simulink model "model"  (R2026b)
settings: Solver=VariableStepAuto  StopTime=5.5  FixedStep=0.0001
InitFcn:
  | init_vehicle;
values from neighbouring files (symbols this model uses):
  vehicle = Simulink.Parameter(vehicle)    [fit_log.m]    (also in init_vehicle.m)
undefined symbols (not defined in the file or in its folder): b6bc
libraries: simulink x2, slpidlib x1
settings Model: Creator=Madelyn  LastModifiedBy=Madelyn
settings RTWCC: GPUComputeCapability=5.0

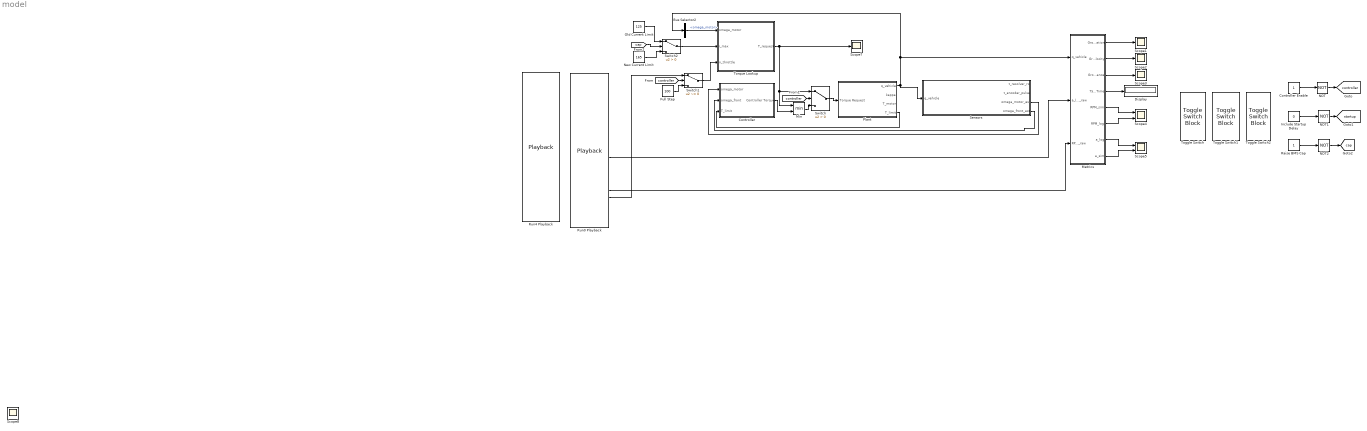
== system model ==
  Bus Selector2 : BusSelector  OutputSignals=omega_motor
  Controller : Subsystem
  Controller Enable : Constant
  Display : Display
  Full Step : Constant  Value=100
  Include Startup Delay : Constant  Value=0
  Metrics : Subsystem
  Min : MinMax  Inputs=2
  NOT : Logic  Operator=NOT  IconShape=distinctive  AllPortsSameDT=off  OutDataTypeStr=boolean
  NOT1 : Logic  Operator=NOT  IconShape=distinctive  AllPortsSameDT=off  OutDataTypeStr=boolean
  NOT2 : Logic  Operator=NOT  IconShape=distinctive  AllPortsSameDT=off  OutDataTypeStr=boolean
  New Current Limit : Constant  Value=165
  Old Current Limit : Constant  Value=125
  Plant : Subsystem
  Raise BMS Cap : Constant
  Run0 Playback : Playback  NumPorts=35  PartName=7320df4f-afde-441e-80d8-dbf4e5708069  TablePosition=Bottom
  Run4 Playback : Playback  NumPorts=35  PartName=9ae1c79e-69de-485c-b6bc-1278a8bcc222  TablePosition=Bottom
  Scope{1..3,7..8} (5 alike) : Scope
      Scope1 settings: ActiveDisplayYMinimum=-1.0070209667799948  ActiveDisplayYMaximum=9.0631887010199552
      Scope2 settings: ActiveDisplayYMinimum=-4.8200936981689466  ActiveDisplayYMaximum=37.977704065737591  DataLoggingVariableName=ScopeData3
      Scope3 settings: DataLoggingVariableName=ScopeData5
      Scope7 settings: ActiveDisplayYMinimum=100.18093555938822  ActiveDisplayYMaximum=233.31322938229022  DataLoggingVariableName=ScopeData11
      Scope8 settings: ActiveDisplayYMinimum=-12.499999999999996  ActiveDisplayYMaximum=112.5  DataLoggingVariableName=ScopeData9
  Scope4 : Scope  NumInputPorts=2
      settings: DataLoggingVariableName=ScopeData7
  Scope5 : Scope  NumInputPorts=2
      settings: DataLoggingVariableName=ScopeData8
  Sensors : Subsystem
  Switch : Switch  Criteria=u2 > Threshold  SaturateOnIntegerOverflow=off  InputSameDT=off
  Switch1 : Switch  Criteria=u2 ~= 0  SaturateOnIntegerOverflow=off  InputSameDT=off
  Switch2 : Switch  Criteria=u2 > Threshold  SaturateOnIntegerOverflow=off  InputSameDT=off
  Toggle Switch : ToggleSwitchBlock
  Toggle Switch1 : ToggleSwitchBlock
  Toggle Switch2 : ToggleSwitchBlock
  Torque Lookup : MATLAB Function  TreatAsAtomicUnit=on
  tag scope: cap=global, controller=global, startup=global
  wires:
  Sensors/3(omega_motor_est) -> Controller/1(omega_motor)
  Sensors/4(omega_front_est) -> Controller/2(omega_front)
  Plant/1(q_vehicle) -> Sensors/1(q_vehicle), Bus Selector2/1, Metrics/1(q_vehicle)
  Bus Selector2/1 -> Torque Lookup/1(omega_motor)  "<omega_motor>"
  Run0 Playback/20 -> Metrics/2(a_log_raw)
  Run0 Playback/29 -> Metrics/3(RPM_log_raw)
  Torque Lookup/1(T_request) -> Scope7/1, Min/1, Switch/1
  Run0 Playback/31 -> Switch1/1
  Min/1 -> Switch/3
  Full Step/1 -> Switch1/3
  Switch1/1 -> Torque Lookup/3(n_throttle)
  Controller Enable/1 -> NOT/1
  [controller] -> Switch1/2
  [controller] -> Switch/2
  NOT/1 -> [controller]
  Include Startup Delay/1 -> NOT1/1
  NOT1/1 -> [startup]
  Raise BMS Cap/1 -> NOT2/1
  NOT2/1 -> [cap]
  Old Current Limit/1 -> Switch2/1
  Switch2/1 -> Torque Lookup/2(i_max)
  New Current Limit/1 -> Switch2/3
  [cap] -> Switch2/2
  Metrics/1(Ground Acceleration) -> Scope1/1
  Metrics/2(Ground Velocity) -> Scope2/1
  Metrics/3(Ground Distance) -> Scope3/1
  Metrics/4(75m Time) -> Display/1
  Metrics/5(RPM_sim) -> Scope4/1
  Metrics/6(RPM_log) -> Scope4/2
  Metrics/7(a_log) -> Scope5/1
  Metrics/8(a_sim) -> Scope5/2
  Controller/1(Controller Torque) -> Min/2
  Plant/4(T_limit) -> Controller/3(T_limit)
  Switch/1 -> Plant/1(Torque Request)

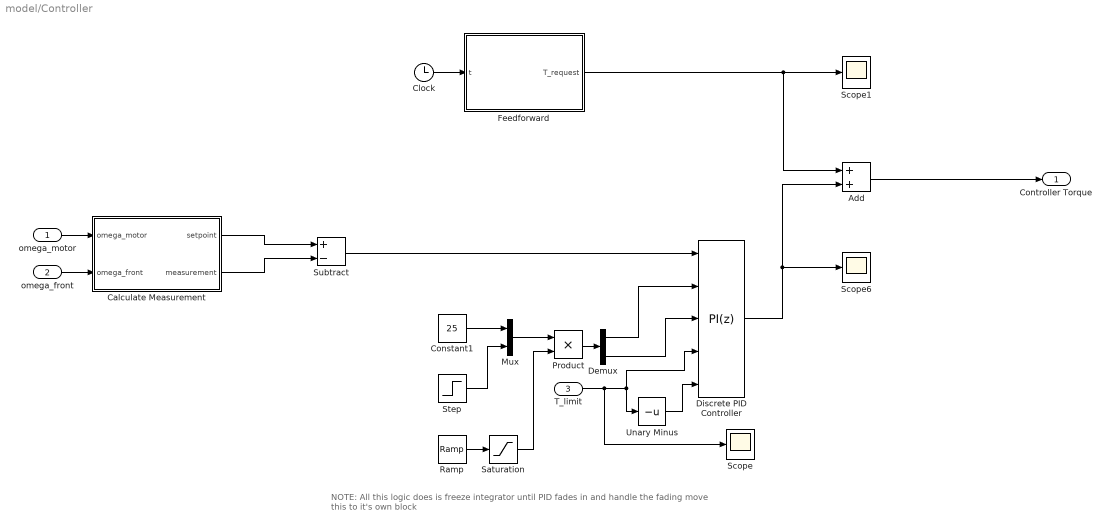
== system model/Controller ==
  note: NOTE: All this logic does is freeze integrator until PID fades in and handle the fading
      | move this to it's own block
  omega_motor : Inport
  omega_front : Inport  Port=2
  T_limit : Inport  Port=3
  Add : Sum
  Calculate Measurement : MATLAB Function  TreatAsAtomicUnit=on
  Clock : Clock
  Constant1 : Constant  Value=25
  Demux : Demux  Outputs=2
  Discrete PID Controller : slpidlib/PID Controller  Controller=PI  Form=Parallel  TimeDomain=Discrete-time  UseExternalTs=off  SampleTime=0.003  IntegratorMethod=Forward Euler  FilterMethod=Forward Euler  ControllerParametersSource=external  P=50  I=400  UseKiTs=off  D=0  UseExternalDerivativeSource=off  N=100  UseFilter=on  TunerSelectOption=Transfer Function Based (PID Tuner App)  InitialConditionSource=internal  InitialConditionForIntegrator=0  InitialConditionForFilter=0  DifferentiatorICPrevScaledInput=0  ExternalReset=none  TrackingMode=off  Kt=1  LimitOutput=on  SatLimitsSource=external  UpperSaturationLimit=inf  LowerSaturationLimit=-inf  LinearizeAsGain=off  AntiWindupMode=clamping  Kb=1  LimitIntegrator=on  UpperIntegratorSaturationLimit=180  LowerIntegratorSaturationLimit=-180  POutMin=[]  POutMax=[]  IOutMin=[]  IOutMax=[]  DOutMin=[]  DOutMax=[]  NOutMin=[]  NOutMax=[]  SumOutMin=[]  SumOutMax=[]  SaturationOutMin=[]  SaturationOutMax=[]  PParamMin=[]  PParamMax=[]  IParamMin=[]  IParamMax=[]  DParamMin=[]  DParamMax=[]  NParamMin=[]  NParamMax=[]  KbParamMin=[]  KbParamMax=[]  KtParamMin=[]  KtParamMax=[]  KbOutMin=[]  KbOutMax=[]  KtOutMin=[]  KtOutMax=[]  IntegratorOutMin=[]  IntegratorOutMax=[]  FilterOutMin=[]  FilterOutMax=[]  SumI1OutMin=[]  SumI1OutMax=[]  SumI2OutMin=[]  SumI2OutMax=[]  SumI3OutMin=[]  SumI3OutMax=[]  SumI4OutMin=[]  SumI4OutMax=[]  SumDOutMin=[]  SumDOutMax=[]  DifferentiatorOutMin=[]  DifferentiatorOutMax=[]  FilterDiffOutCoefMin=[]  FilterDiffOutCoefMax=[]  ReciprocalOutMin=[]  ReciprocalOutMax=[]  SumDenOutMin=[]  SumDenOutMax=[]  SumNumOutMin=[]  SumNumOutMax=[]  DivideOutMin=[]  DivideOutMax=[]  UdiffTsProdOutMin=[]  UdiffTsProdOutMax=[]  NTsProdOutMin=[]  NTsProdOutMax=[]  UintegralTsProdOutMin=[]  UintegralTsProdOutMax=[]  UngainTsProdOutMin=[]  UngainTsProdOutMax=[]  ClampingZeroOutDataTypeStr=Inherit: Inherit via back propagation  ClampingZeroOutMin=[]  ClampingZeroOutMax=[]  FilterDenConstantOutDataTypeStr=Inherit: Inherit via back propagation  FilterDenConstantOutMin=[]  FilterDenConstantOutMax=[]  PCopyOutDataTypeStr=Inherit: Inherit via back propagation  PCopyOutMin=[]  PCopyOutMax=[]  NCopyOutDataTypeStr=Inherit: Inherit via back propagation  NCopyOutMin=[]  NCopyOutMax=[]  IntegratorContinuousStateAttributes=''  IntegratorStateMustResolveToSignalObject=off  IntegratorRTWStateStorageClass=Auto  FilterContinuousStateAttributes=''  FilterStateMustResolveToSignalObject=off  FilterRTWStateStorageClass=Auto  ParallelPVariant=ExternalParameters  IdealPVariant=Disabled  IVariant=ExternalParameters  DVariant=Disabled  IntegratorVariant=Discrete  SatVariant=External  AWVariant=DiscClampingParallel  PCopyVariant=Disabled  TRVariant=Disabled  FdbkBlocksVariant=Forward  IdealPFdbkVariant=Disabled  SatFdbkVariant=Disabled  DerivativeFilterVariant=Disabled  NVariant=Disabled  NCopyVariant=Disabled_SignalSpec  FilterICVariant=Disabled  IntegratorICVariant=InternalICs  ExternalResetVariant=Disabled  TRSumVariant=Passthrough  SumFdbkVariant=Disabled  SumVariant=Sum_PI  TsampFilterVariant=InternalTs  TsampNgainVariant=Passthrough  TsampIntegralVariant=Disabled_SignalSpec  ExternalSaturationOutDataTypeStr=Inherit: Same as second input  DerivativeSourceVariant=Disabled  PreIntVariant=InternalPreInt
      settings: LibrarySourceBlock=simulink/Discrete/Discrete PID Controller
  Feedforward : MATLAB Function  TreatAsAtomicUnit=on
  Mux : Mux  Inputs=2
  Product : Product
  Ramp : simulink/Sources/Ramp  slope=4  start=0.5  InitialOutput=0
  Saturation : Saturate  UpperLimit=1  LowerLimit=0
  Scope : Scope
      settings: ActiveDisplayYMinimum=130.59305560506354  ActiveDisplayYMaximum=189.48966048832625  DataLoggingVariableName=ScopeData16
  Scope1 : Scope
      settings: ActiveDisplayYMinimum=-19.769298544681185  ActiveDisplayYMaximum=177.9236869021307
  Scope6 : Scope
      settings: ActiveDisplayYMinimum=-24.158543429115252  ActiveDisplayYMaximum=189.40218177528487  DataLoggingVariableName=ScopeData6
  Step : Step  Time=0.5  FinalValue=250  SampleTime=0
  Subtract : Sum  Inputs=+-
  Unary Minus : UnaryMinus
  Controller Torque : Outport
  wires:
  Ramp/1 -> Saturation/1
  Mux/1 -> Product/1
  Constant1/1 -> Mux/1
  Product/1 -> Demux/1
  Saturation/1 -> Product/2
  Feedforward/1(T_request) -> Add/1, Scope1/1
  Step/1 -> Mux/2
  Demux/1 -> Discrete PID Controller/2
  Demux/2 -> Discrete PID Controller/3
  Add/1 -> Controller Torque/1
  T_limit/1 -> Scope/1, Unary Minus/1, Discrete PID Controller/4
  Unary Minus/1 -> Discrete PID Controller/5
  Discrete PID Controller/1 -> Scope6/1, Add/2
  omega_motor/1 -> Calculate Measurement/1(omega_motor)
  omega_front/1 -> Calculate Measurement/2(omega_front)
  Subtract/1 -> Discrete PID Controller/1
  Calculate Measurement/1(setpoint) -> Subtract/1
  Calculate Measurement/2(measurement) -> Subtract/2
  Clock/1 -> Feedforward/1(t)

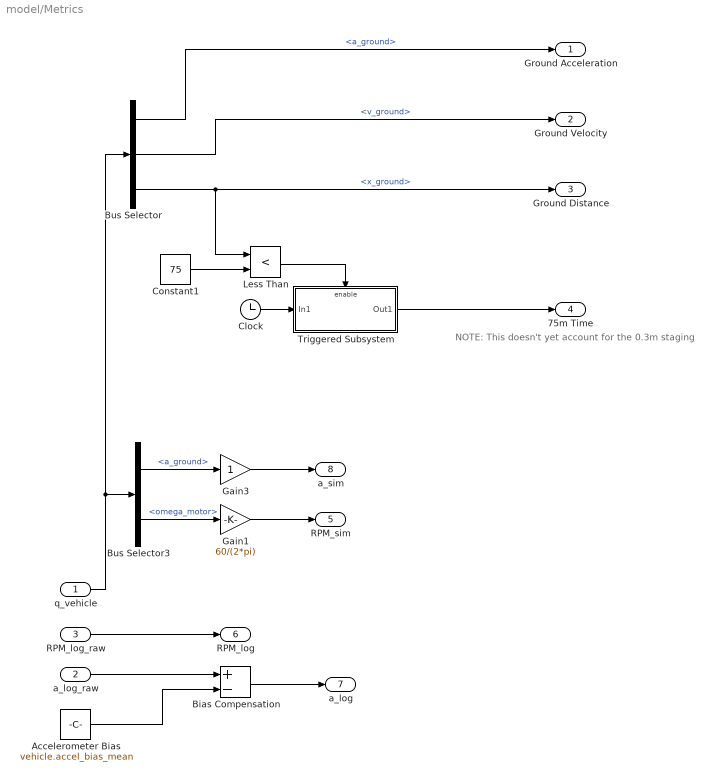
== system model/Metrics ==
  note: NOTE: This doesn't yet account for the 0.3m staging
  q_vehicle : Inport
  a_log_raw : Inport  Port=2
  RPM_log_raw : Inport  Port=3
  Accelerometer Bias : Constant  Value=vehicle.accel_bias_mean
  Bias Compensation : Sum  Inputs=+-
  Bus Selector : BusSelector  OutputSignals=a_ground,v_ground,x_ground
  Bus Selector3 : BusSelector  OutputSignals=a_ground,omega_motor
  Clock : Clock
  Constant1 : Constant  Value=75
  Gain1 : Gain  Gain=60/(2*pi)
  Gain3 : Gain
  Less Than : RelationalOperator  Operator=<  OutDataTypeStr=boolean  RndMeth=Simplest  InputSameDT=off
  Triggered Subsystem : Subsystem  TreatAsAtomicUnit=on
  Ground Acceleration : Outport
  Ground Velocity : Outport  Port=2
  Ground Distance : Outport  Port=3
  75m Time : Outport  Port=4
  RPM_sim : Outport  Port=5
  RPM_log : Outport  Port=6
  a_log : Outport  Port=7
  a_sim : Outport  Port=8
  wires:
  RPM_log_raw/1 -> RPM_log/1
  Accelerometer Bias/1 -> Bias Compensation/2
  a_log_raw/1 -> Bias Compensation/1
  Bus Selector3/1 -> Gain3/1  "<a_ground>"
  Gain1/1 -> RPM_sim/1
  q_vehicle/1 -> Bus Selector/1, Bus Selector3/1
  Bus Selector/2 -> Ground Velocity/1  "<v_ground>"
  Constant1/1 -> Less Than/2
  Less Than/1 -> Triggered Subsystem/Enable
  Bus Selector/3 -> Ground Distance/1, Less Than/1  "<x_ground>"
  Clock/1 -> Triggered Subsystem/1(In1)
  Bus Selector/1 -> Ground Acceleration/1  "<a_ground>"
  Bus Selector3/2 -> Gain1/1  "<omega_motor>"
  Triggered Subsystem/1(Out1) -> 75m Time/1
  Bias Compensation/1 -> a_log/1
  Gain3/1 -> a_sim/1

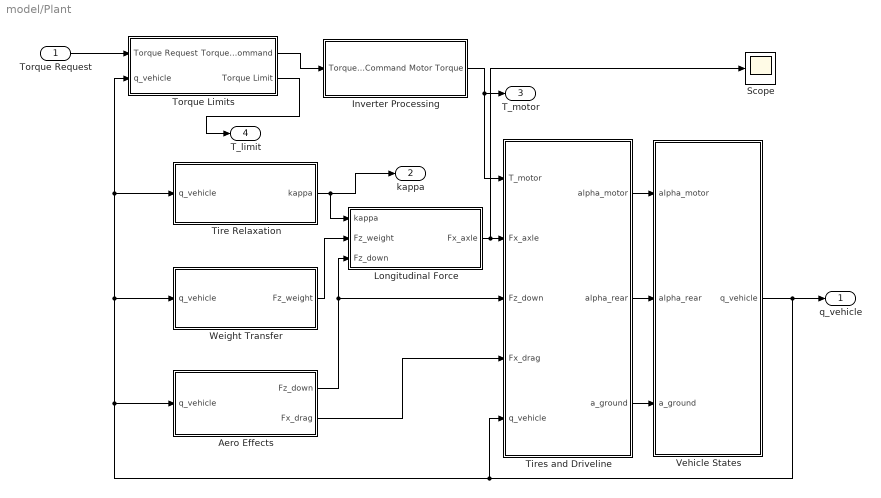
== system model/Plant ==
  Torque Request : Inport
  Aero Effects : Subsystem
  Inverter Processing : Subsystem
  Longitudinal Force : Subsystem
  Scope : Scope
      settings: ActiveDisplayYMinimum=-349.40408874349123  ActiveDisplayYMaximum=3144.6367986914215  DataLoggingVariableName=ScopeData4
  Tire Relaxation : Subsystem
  Tires and Driveline : Subsystem
  Torque Limits : Subsystem
  Vehicle States : Subsystem
  Weight Transfer : Subsystem
  q_vehicle : Outport
  kappa : Outport  Port=2
  T_motor : Outport  Port=3
  T_limit : Outport  Port=4
  wires:
  Tires and Driveline/3(a_ground) -> Vehicle States/3(a_ground)
  Vehicle States/1(q_vehicle) -> Tire Relaxation/1(q_vehicle), Torque Limits/2(q_vehicle), Weight Transfer/1(q_vehicle), Aero Effects/1(q_vehicle), Tires and Driveline/5(q_vehicle), q_vehicle/1
  Tires and Driveline/2(alpha_rear) -> Vehicle States/2(alpha_rear)
  Tires and Driveline/1(alpha_motor) -> Vehicle States/1(alpha_motor)
  Torque Limits/1(Torque Command) -> Inverter Processing/1(Torque Command)
  Tire Relaxation/1(kappa) -> kappa/1, Longitudinal Force/1(kappa)
  Weight Transfer/1(Fz_weight) -> Longitudinal Force/2(Fz_weight)
  Longitudinal Force/1(Fx_axle) -> Scope/1, Tires and Driveline/2(Fx_axle)
  Inverter Processing/1(Motor Torque) -> T_motor/1, Tires and Driveline/1(T_motor)
  Torque Request/1 -> Torque Limits/1(Torque Request)
  Torque Limits/2(Torque Limit) -> T_limit/1
  Aero Effects/2(Fx_drag) -> Tires and Driveline/4(Fx_drag)
  Aero Effects/1(Fz_down) -> Tires and Driveline/3(Fz_down), Longitudinal Force/3(Fz_down)

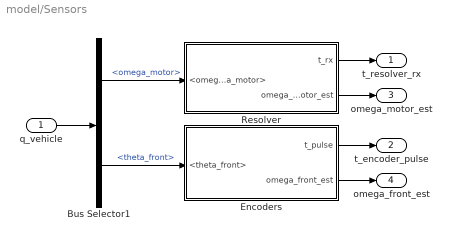
== system model/Sensors ==
  q_vehicle : Inport
  Bus Selector1 : BusSelector  OutputSignals=omega_motor,theta_front
  Encoders : Subsystem
  Resolver : Subsystem
  t_resolver_rx : Outport
  t_encoder_pulse : Outport  Port=2
  omega_motor_est : Outport  Port=3
  omega_front_est : Outport  Port=4
  wires:
  Bus Selector1/2 -> Encoders/1(<theta_front>)  "<theta_front>"
  q_vehicle/1 -> Bus Selector1/1
  Bus Selector1/1 -> Resolver/1(<omega_motor>)  "<omega_motor>"
  Resolver/1(t_rx) -> t_resolver_rx/1
  Resolver/2(omega_motor_est) -> omega_motor_est/1
  Encoders/1(t_pulse) -> t_encoder_pulse/1
  Encoders/2(omega_front_est) -> omega_front_est/1

== system model/Metrics/Triggered Subsystem ==
  In1 : Inport
  Enable : EnablePort
  Out1 : Outport
  wires:
  In1/1 -> Out1/1

== system model/Plant/Aero Effects ==
  q_vehicle : Inport
  Aero Effects : MATLAB Function  TreatAsAtomicUnit=on
  Bus Selector : BusSelector  OutputSignals=v_ground
  Fz_down : Outport
  Fx_drag : Outport  Port=2
  wires:
  Bus Selector/1 -> Aero Effects/1(v_ground)  "<v_ground>"
  q_vehicle/1 -> Bus Selector/1
  Aero Effects/1(Fz_down) -> Fz_down/1
  Aero Effects/2(Fx_drag) -> Fx_drag/1

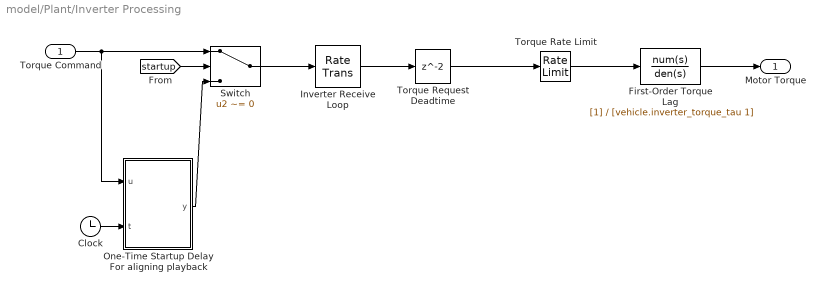
== system model/Plant/Inverter Processing ==
  Torque Command : Inport
  Clock : Clock
  First-Order Torque Lag : TransferFcn  Denominator=[vehicle.inverter_torque_tau 1]
  Inverter Receive Loop : RateTransition  OutPortSampleTime=vehicle.inverter_receive_period
  One-Time Startup Delay For aligning playback : MATLAB Function  TreatAsAtomicUnit=on
  Switch : Switch  Criteria=u2 ~= 0  SaturateOnIntegerOverflow=off  InputSameDT=off
  Torque Rate Limit : RateLimiter  RisingSlewLimit=vehicle.torque_rate_limit  FallingSlewLimit=-vehicle.torque_rate_limit  SampleTimeMode=inherited
  Torque Request Deadtime : Delay  SampleTime=vehicle.inverter_request_deadtime
  Motor Torque : Outport
  wires:
  Torque Rate Limit/1 -> First-Order Torque Lag/1
  Inverter Receive Loop/1 -> Torque Request Deadtime/1
  First-Order Torque Lag/1 -> Motor Torque/1
  Torque Request Deadtime/1 -> Torque Rate Limit/1
  Clock/1 -> One-Time Startup Delay For aligning playback/2(t)
  Torque Command/1 -> One-Time Startup Delay For aligning playback/1(u), Switch/1
  One-Time Startup Delay For aligning playback/1(y) -> Switch/3
  Switch/1 -> Inverter Receive Loop/1
  [startup] -> Switch/2

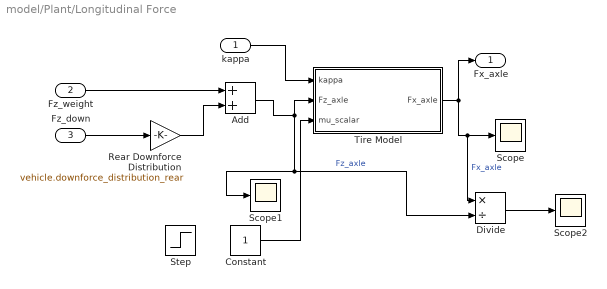
== system model/Plant/Longitudinal Force ==
  kappa : Inport
  Fz_weight : Inport  Port=2
  Fz_down : Inport  Port=3
  Add : Sum
  Constant : Constant
  Divide : Product  Inputs=*/
  "Rear Downforce Distribution " : Gain  Gain=vehicle.downforce_distribution_rear
  Scope : Scope
      settings: ActiveDisplayYMinimum=-328.964155800479  ActiveDisplayYMaximum=2960.6774022043114  DataLoggingVariableName=ScopeData13
  Scope1 : Scope
      settings: ActiveDisplayYMinimum=1302.8307308940846  ActiveDisplayYMaximum=2187.5559219532392  DataLoggingVariableName=ScopeData14
  Scope2 : Scope
      settings: ActiveDisplayYMinimum=-0.1766422510137696  ActiveDisplayYMaximum=1.5897802591239265  DataLoggingVariableName=ScopeData15
  Step : Step  Time=1.5  InitialValue=1  FinalValue=0.8  SampleTime=0
  Tire Model : MATLAB Function  TreatAsAtomicUnit=on
  Fx_axle : Outport
  wires:
  Fz_down/1 -> "Rear Downforce Distribution "/1
  kappa/1 -> Tire Model/1(kappa)
  Add/1 -> Divide/2, Scope1/1, Tire Model/2(Fz_axle)  "Fz_axle"
  Fz_weight/1 -> Add/1
  "Rear Downforce Distribution "/1 -> Add/2
  Tire Model/1(Fx_axle) -> Fx_axle/1, Divide/1, Scope/1  "Fx_axle"
  Divide/1 -> Scope2/1
  Constant/1 -> Tire Model/3(mu_scalar)

== system model/Plant/Tire Relaxation ==
  q_vehicle : Inport
  Bus Selector : BusSelector  OutputSignals=omega_rear,v_ground
  Integrator : Integrator
  Saturation1 : Saturate  UpperLimit=vehicle.tire_relaxation_length*vehicle.kappa_max  LowerLimit=-vehicle.tire_relaxation_length*vehicle.kappa_max
  Tire Relaxation : MATLAB Function  TreatAsAtomicUnit=on
  kappa : Outport
  wires:
  Tire Relaxation/1(kappa) -> kappa/1
  Tire Relaxation/2(udot) -> Integrator/1
  Integrator/1 -> Saturation1/1
  Saturation1/1 -> Tire Relaxation/3(u)
  q_vehicle/1 -> Bus Selector/1
  Bus Selector/2 -> Tire Relaxation/2(v_ground)  "<v_ground>"
  Bus Selector/1 -> Tire Relaxation/1(omega_rear)  "<omega_rear>"

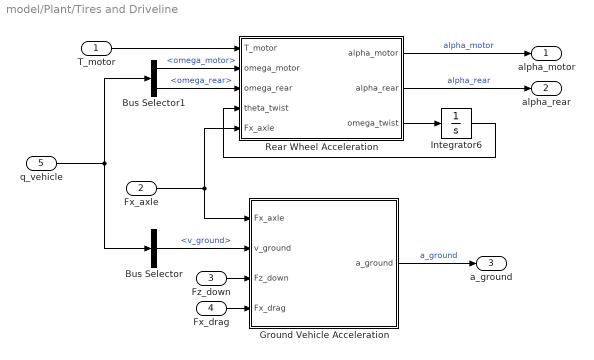
== system model/Plant/Tires and Driveline ==
  T_motor : Inport
  Fx_axle : Inport  Port=2
  Fz_down : Inport  Port=3
  Fx_drag : Inport  Port=4
  q_vehicle : Inport  Port=5
  Bus Selector : BusSelector  OutputSignals=v_ground
  Bus Selector1 : BusSelector  OutputSignals=omega_motor,omega_rear
  Ground Vehicle Acceleration : MATLAB Function  TreatAsAtomicUnit=on
  Integrator6 : Integrator
  Rear Wheel Acceleration : MATLAB Function  TreatAsAtomicUnit=on
  alpha_motor : Outport
  alpha_rear : Outport  Port=2
  a_ground : Outport  Port=3
  wires:
  Ground Vehicle Acceleration/1(a_ground) -> a_ground/1  "a_ground"
  Bus Selector/1 -> Ground Vehicle Acceleration/2(v_ground)  "<v_ground>"
  Bus Selector1/1 -> Rear Wheel Acceleration/2(omega_motor)  "<omega_motor>"
  Rear Wheel Acceleration/3(omega_twist) -> Integrator6/1
  Bus Selector1/2 -> Rear Wheel Acceleration/3(omega_rear)  "<omega_rear>"
  Integrator6/1 -> Rear Wheel Acceleration/4(theta_twist)
  T_motor/1 -> Rear Wheel Acceleration/1(T_motor)
  Rear Wheel Acceleration/2(alpha_rear) -> alpha_rear/1  "alpha_rear"
  Rear Wheel Acceleration/1(alpha_motor) -> alpha_motor/1  "alpha_motor"
  Fx_drag/1 -> Ground Vehicle Acceleration/4(Fx_drag)
  Fx_axle/1 -> Ground Vehicle Acceleration/1(Fx_axle), Rear Wheel Acceleration/5(Fx_axle)
  Fz_down/1 -> Ground Vehicle Acceleration/3(Fz_down)
  q_vehicle/1 -> Bus Selector1/1, Bus Selector/1

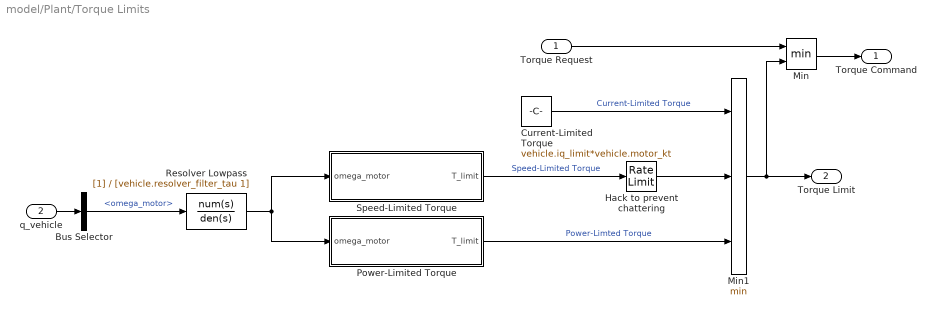
== system model/Plant/Torque Limits ==
  Torque Request : Inport
  q_vehicle : Inport  Port=2
  " Power-Limited Torque" : MATLAB Function  TreatAsAtomicUnit=on
  Bus Selector : BusSelector  OutputSignals=omega_motor
  Current-Limited Torque : Constant  Value=vehicle.iq_limit*vehicle.motor_kt
  Hack to prevent chattering : RateLimiter  RisingSlewLimit=200  FallingSlewLimit=-200  SampleTimeMode=inherited
  Min : MinMax  Inputs=2
  Min1 : MinMax  Inputs=3
  Resolver Lowpass : TransferFcn  Denominator=[vehicle.resolver_filter_tau 1]
  Speed-Limited Torque : MATLAB Function  TreatAsAtomicUnit=on
  Torque Command : Outport
  Torque Limit : Outport  Port=2
  wires:
  Current-Limited Torque/1 -> Min1/1  "Current-Limited Torque"
  " Power-Limited Torque"/1(T_limit) -> Min1/3  "Power-Limted Torque"
  Torque Request/1 -> Min/1
  Bus Selector/1 -> Resolver Lowpass/1  "<omega_motor>"
  q_vehicle/1 -> Bus Selector/1
  Speed-Limited Torque/1(T_limit) -> Hack to prevent chattering/1  "Speed-Limited Torque"
  Resolver Lowpass/1 -> " Power-Limited Torque"/1(omega_motor), Speed-Limited Torque/1(omega_motor)
  Hack to prevent chattering/1 -> Min1/2
  Min1/1 -> Torque Limit/1, Min/2
  Min/1 -> Torque Command/1

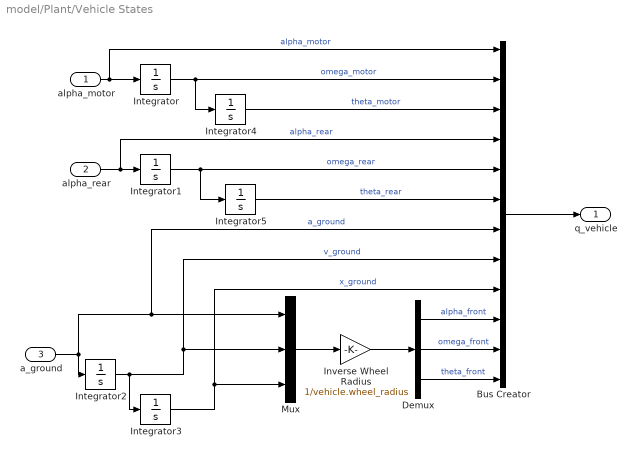
== system model/Plant/Vehicle States ==
  alpha_motor : Inport
  alpha_rear : Inport  Port=2
  a_ground : Inport  Port=3
  Bus Creator : BusCreator  Inputs=12
  Demux : Demux  Outputs=3
  Integrator{,1..5} (6 alike) : Integrator
  Inverse Wheel Radius : Gain  Gain=1/vehicle.wheel_radius
  Mux : Mux  Inputs=3
  q_vehicle : Outport
  wires:
  alpha_rear/1 -> Bus Creator/4, Integrator1/1  "alpha_rear"
  a_ground/1 -> Integrator2/1, Bus Creator/7, Mux/1  "a_ground"
  Demux/1 -> Bus Creator/10  "alpha_front"
  Integrator3/1 -> Bus Creator/9, Mux/3  "x_ground"
  Mux/1 -> Inverse Wheel Radius/1
  Integrator/1 -> Bus Creator/2, Integrator4/1  "omega_motor"
  Integrator2/1 -> Integrator3/1, Bus Creator/8, Mux/2  "v_ground"
  Integrator4/1 -> Bus Creator/3  "theta_motor"
  Demux/3 -> Bus Creator/12  "theta_front"
  alpha_motor/1 -> Bus Creator/1, Integrator/1  "alpha_motor"
  Integrator1/1 -> Bus Creator/5, Integrator5/1  "omega_rear"
  Integrator5/1 -> Bus Creator/6  "theta_rear"
  Demux/2 -> Bus Creator/11  "omega_front"
  Inverse Wheel Radius/1 -> Demux/1
  Bus Creator/1 -> q_vehicle/1

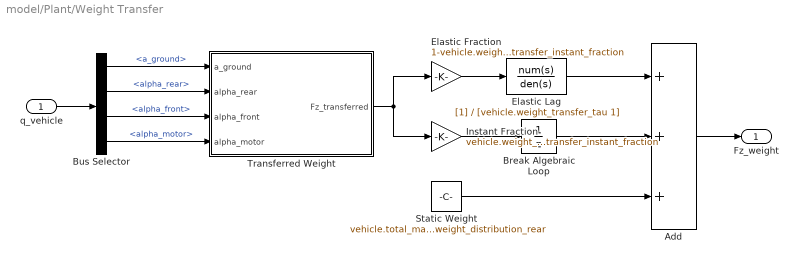
== system model/Plant/Weight Transfer ==
  q_vehicle : Inport
  Add : Sum  Inputs=+++
  Break Algebraic Loop : UnitDelay  SampleTime=-1
  Bus Selector : BusSelector  OutputSignals=a_ground,alpha_rear,alpha_front,alpha_motor
  Elastic Fraction : Gain  Gain=1-vehicle.weight_transfer_instant_fraction
  Elastic Lag : TransferFcn  Denominator=[vehicle.weight_transfer_tau 1]
  Instant Fraction : Gain  Gain=vehicle.weight_transfer_instant_fraction
  Static Weight : Constant  Value=vehicle.total_mass*vehicle.gravity_acceleration*vehicle.weight_distribution_rear
  Transferred Weight : MATLAB Function  TreatAsAtomicUnit=on
  Fz_weight : Outport
  wires:
  Elastic Fraction/1 -> Elastic Lag/1
  Add/1 -> Fz_weight/1
  Instant Fraction/1 -> Break Algebraic Loop/1
  Transferred Weight/1(Fz_transferred) -> Instant Fraction/1, Elastic Fraction/1
  Elastic Lag/1 -> Add/1
  Break Algebraic Loop/1 -> Add/2
  q_vehicle/1 -> Bus Selector/1
  Static Weight/1 -> Add/3
  Bus Selector/1 -> Transferred Weight/1(a_ground)  "<a_ground>"
  Bus Selector/2 -> Transferred Weight/2(alpha_rear)  "<alpha_rear>"
  Bus Selector/3 -> Transferred Weight/3(alpha_front)  "<alpha_front>"
  Bus Selector/4 -> Transferred Weight/4(alpha_motor)  "<alpha_motor>"

== system model/Sensors/Encoders ==
  <theta_front> : Inport
  Clock1 : Clock
  Encoder Quantization : MATLAB Function  TreatAsAtomicUnit=on
  Unit Delay : UnitDelay  SampleTime=-1
  Unit Delay1 : UnitDelay  SampleTime=-1
  t_pulse : Outport
  omega_front_est : Outport  Port=2
  wires:
  Clock1/1 -> Unit Delay1/1, Encoder Quantization/3(t)
  Unit Delay/1 -> Encoder Quantization/2(pos_prev)
  Encoder Quantization/2(t_pulse) -> t_pulse/1
  <theta_front>/1 -> Encoder Quantization/1(pos), Unit Delay/1
  Unit Delay1/1 -> Encoder Quantization/4(t_prev)
  Encoder Quantization/1(omega_front_est) -> omega_front_est/1

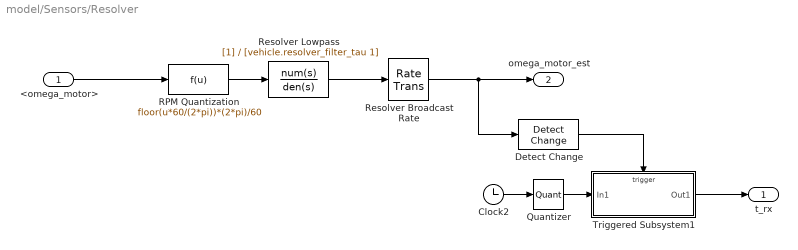
== system model/Sensors/Resolver ==
  <omega_motor> : Inport
  Clock2 : Clock
  Detect Change : simulink/Logic and Bit Operations/Detect Change  vinit=0  OutDataTypeStr=boolean
  Quantizer : Quantizer  QuantizationInterval=1/1000
  RPM Quantization : Fcn  Expr=floor(u*60/(2*pi))*(2*pi)/60
  Resolver Broadcast Rate : RateTransition  OutPortSampleTime=vehicle.inverter_transmit_period
  Resolver Lowpass : TransferFcn  Denominator=[vehicle.resolver_filter_tau 1]
  Triggered Subsystem1 : Subsystem  TreatAsAtomicUnit=on
  t_rx : Outport
  omega_motor_est : Outport  Port=2
  wires:
  Detect Change/1 -> Triggered Subsystem1/Trigger
  RPM Quantization/1 -> Resolver Lowpass/1
  Resolver Lowpass/1 -> Resolver Broadcast Rate/1
  Clock2/1 -> Quantizer/1
  Resolver Broadcast Rate/1 -> Detect Change/1, omega_motor_est/1
  <omega_motor>/1 -> RPM Quantization/1
  Quantizer/1 -> Triggered Subsystem1/1(In1)
  Triggered Subsystem1/1(Out1) -> t_rx/1

== system model/Sensors/Resolver/Triggered Subsystem1 ==
  In1 : Inport
  Trigger : TriggerPort  VariantControl=(inherit)
  Out1 : Outport
  wires:
  In1/1 -> Out1/1

== matlab function model/Torque Lookup ==
  data: omega_motor input; T_request output; i_max input; n_throttle input; vehicle parameter
function T_request = fcn(omega_motor, i_max, n_throttle, vehicle)
    motor_speed = omega_motor * 60/(2*pi);
    current_limit = i_max;

    torque_limit_local = min(vehicle.motor_torque_limit, vehicle.nominal_battery_voltage * current_limit / max(230.4, motor_speed * 0.1076));
    
    if motor_speed >= 6000
        torque_limit_local = 30;
    end
    
    T_request = n_throttle/100 * torque_limit_local;
end

== matlab function model/Plant/Inverter Processing/One-Time Startup Delay For aligning playback ==
  settings: updateMethod=DISCRETE
  data: u input; y output; t input; vehicle parameter
function y = fcn(u, t, vehicle)
    persistent t_initial triggered;
    
    if isempty(triggered)
        t_initial = 0;
        triggered = false;
    end
    
    if ~triggered && (u ~= 0)
        triggered = true;
        t_initial = t; 
    end
    
    if triggered && (t >= t_initial + vehicle.launch_startup_delay)
        y = u;
    else
        y = 0;
    end
end

== matlab function model/Plant/Aero Effects/Aero Effects ==
  data: Fz_down output; v_ground input; Fx_drag output; vehicle parameter
function [Fz_down, Fx_drag] = fcn(v_ground, vehicle)
    q_signed = 0.5*vehicle.air_density*v_ground*abs(v_ground);
    q_pos    = 0.5*vehicle.air_density*v_ground^2;
    
    Fx_drag = q_signed*vehicle.drag_coefficient*vehicle.frontal_area;
    Fz_down = q_pos*vehicle.downforce_coefficient*vehicle.frontal_area;
end

== matlab function model/Controller/Calculate Measurement ==
  data: setpoint output; omega_motor input; measurement output; omega_front input; vehicle parameter
function [setpoint, measurement]  = fcn(omega_motor, omega_front, vehicle)
    kappa=0.12;
    v_front=omega_front*vehicle.wheel_radius;
    setpoint=v_front*kappa;
    measurement=(omega_motor * 1/vehicle.gear_ratio * vehicle.wheel_radius - v_front);
end

== matlab function model/Plant/Torque Limits/ Power-Limited Torque ==
  data: omega_motor input; T_limit output; vehicle parameter
function T_limit = fcn(omega_motor, vehicle)
    T_limit = vehicle.gearbox_efficiency * vehicle.power_limit/max(abs(omega_motor), 0.5);
end

== matlab function model/Plant/Torque Limits/Speed-Limited Torque ==
  data: omega_motor input; T_limit output; vehicle parameter
function T_limit = fcn(omega_motor, vehicle)
    rpm   = omega_motor*60/(2*pi);
    w0    = vehicle.motor_speed_limit;
    ramp  = (1.02*w0 - rpm) / (0.02*w0);       % 1 below w0, 0 above 1.02*w0
    T_limit = vehicle.motor_torque_limit * min(max(ramp, 0), 1);
end

== matlab function model/Plant/Tires and Driveline/Rear Wheel Acceleration ==
  data: alpha_motor output; T_motor input; omega_motor input; omega_rear input; theta_twist input; alpha_rear output; Fx_axle input; vehicle parameter; omega_twist output
function [alpha_motor, alpha_rear, omega_twist] = fcn(T_motor, omega_motor, omega_rear, theta_twist, Fx_axle, vehicle)
    % Motor and rear wheel acceleration in mass-spring-mass system

    % reflect to wheel side
    omega_motor_wheelside = omega_motor / vehicle.gear_ratio;
    omega_rear_wheelside = omega_rear;

    % reaction torque from the shafts at the wheel side
    % mass-spring-mass system with damping
    omega_twist=omega_motor_wheelside - omega_rear_wheelside;
    T_shaft  = vehicle.shaft_stiffness*theta_twist + vehicle.shaft_damping*omega_twist;

    % NOTE: rolling resistance is accounted for in the
    % body acceleration block rather than here

    % under acceleration rotor sees:
    % positive driving torque from the motor
    % resistive reaction torque through shafts
    dir=tanh((T_motor * omega_motor) / 20);
    eta=vehicle.gearbox_efficiency^(-dir);
    alpha_motor_wheelside = (vehicle.gear_ratio*T_motor - T_shaft*eta)/vehicle.rotor_inertia_wheelside;

    % under acceleration wheel sees:
    % positive driving torque through shafts
    % resistive reaction torque from road pushing back against tire
    alpha_rear_wheelside=(T_shaft - vehicle.wheel_radius * Fx_axle)/(2*vehicle.wheel_inertia);

    alpha_motor = alpha_motor_wheelside * vehicle.gear_ratio;
    alpha_rear = alpha_rear_wheelside;
end

== matlab function model/Plant/Longitudinal Force/Tire Model ==
  data: kappa input; Fx_axle output; Fz_axle input; mu_scalar input; vehicle parameter
function Fx_axle = fcn(kappa, Fz_axle, mu_scalar, vehicle)
    C = vehicle.tire_C;
    B = vehicle.tire_B;
    E = vehicle.tire_E;
    
    Bx    = B * kappa;
    arg   = Bx - E * (Bx - atan(Bx));
    shape = sin(C * atan(arg));
    
    Fz_tire = max(Fz_axle, 0.0) / 2.0;
    dfz     = (Fz_tire - vehicle.tire_nominal_Fz) / vehicle.tire_nominal_Fz;
    mu_load = mu_scalar * max(vehicle.tire_mu_peak * (1.0 - vehicle.tire_load_sens * dfz), 0.0);
    
    m    = max(min(vehicle.tire_lr_mismatch, 0.99), -0.99);
    mu_l = mu_load * (1.0 + m);
    mu_r = mu_load * (1.0 - m);
    
    if vehicle.open_diff
        Fx_axle = 2.0 * Fz_tire * min(mu_l, mu_r) * shape;
    else
        Fx_axle = Fz_tire * (mu_l + mu_r) * shape;
    end
end

== matlab function model/Plant/Tires and Driveline/Ground Vehicle Acceleration ==
  data: Fx_axle input; a_ground output; v_ground input; Fz_down input; Fx_drag input; vehicle parameter
function a_ground = fcn(Fx_axle, v_ground, Fz_down, Fx_drag, vehicle)
    % Ground vehicle acceleration
    % tanh smoothsign to prevent rolling backwards at 0 velocity
    F_roll=vehicle.rolling_resistance*(vehicle.total_mass*vehicle.gravity_acceleration+Fz_down)*tanh(v_ground/0.1);
    a_ground = (Fx_axle - F_roll - Fx_drag)/(vehicle.total_mass + (2 * vehicle.wheel_inertia)/(vehicle.wheel_radius^2));
end

== matlab function model/Plant/Weight Transfer/Transferred Weight ==
  data: a_ground input; alpha_rear input; alpha_front input; alpha_motor input; Fz_transferred output; vehicle parameter
function Fz_transferred = fcn(a_ground, alpha_rear, alpha_front, alpha_motor, vehicle)
    % Quasi steady state weight transfer fed into first-order lag

    % should these be counted?
    %+ 2*vehicle.wheel_inertia * alpha_rear...
    %+ 2*vehicle.wheel_inertia * alpha_front...
    %+ vehicle.rotor_inertia * alpha_motor...

    Fz_transferred=(...
        vehicle.total_mass*a_ground*vehicle.cg_height...
    )/vehicle.frame_wheelbase;
end

== matlab function model/Plant/Tire Relaxation/Tire Relaxation ==
  data: kappa output; omega_rear input; v_ground input; u input; udot output; vehicle parameter
function [kappa, udot] = fcn(omega_rear, v_ground, u, vehicle)
    % Contact patch deflection tire relaxation
    R     = vehicle.wheel_radius;
    sigma = vehicle.tire_relaxation_length;

    V    = abs(v_ground);
    udot = (R*omega_rear - v_ground) - (V/sigma)*u;
    kappa=u/sigma;
end

== matlab function model/Controller/Feedforward ==
  settings: updateMethod=CONTINUOUS  sampleTime=0.003
  data: T_request output; t input; vehicle parameter
function T_request = fcn(t, vehicle)
    mu_est=1.47;

    Wr = vehicle.total_mass * vehicle.gravity_acceleration * vehicle.weight_distribution_rear;
    F = (mu_est * Wr)/(1 - mu_est * vehicle.cg_height/vehicle.frame_wheelbase);
    
    
    T_hold = (F * vehicle.wheel_radius)/(vehicle.gear_ratio * vehicle.gearbox_efficiency); % fixed point traction limited torque
    T_rate=500;
    T_tau  = 0.125;   % settling time constant for asymptotic approach
    
    T_knee = T_hold - T_rate*T_tau; % force a matching slope to avoid kinks
    t_knee = T_knee / T_rate;
    
    T_request=0;
    if t < 0
        T_request = 0;
    elseif t < t_knee
        T_request = T_rate * t;
    else
        T_request = T_hold - (T_hold - T_knee) * exp(-(t - t_knee)/T_tau);
    end
end

== matlab function model/Sensors/Encoders/Encoder Quantization ==
  settings: updateMethod=DISCRETE
  data: pos input; omega_front_est output; pos_prev input; t input; t_prev input; t_pulse output; vehicle parameter
function [omega_front_est, t_pulse]  = fcn(pos, pos_prev, t, t_prev, vehicle)
    persistent cnt_last target v_last tick_last

    d_theta = (2 * pi)/vehicle.encoder_ppr;

    if isempty(cnt_last)
        cnt_last = 0; target = pos + d_theta; v_last=0; tick_last=0;
    end
    
    Ts = t - t_prev;

    % check if pos has increased enough that it would cause encoder edge
    while Ts > 0 && pos >= target
        % linearly interpolate to find exact* time edge rose
        % NOTE*: assumes constant change between pos and pos_prev!
        % this is probably fine for FSAE accelerations at 100us step
        t_edge = t_prev + (target - pos_prev)/(pos - pos_prev)*Ts;
        
        % quantize to 1MHz tick
        cnt = floor(t_edge/1e-6);
        
        % calculate period
        dT  = cnt - cnt_last;

        % period measurement to velocity
        v_last = d_theta / (dT*1e-6);
        tick_last = cnt;

        % update states
        cnt_last = cnt;
        target = target + d_theta;
    end

    % TODO 0 velocity timeout

    omega_front_est = v_last;
    t_pulse = tick_last;
end
